simulink model "num2ASCIIsequenced_V2"  (Simulink 7.1)
settings: Solver=FixedStepDiscrete  StartTime=0.0  StopTime=.1  FixedStep=.0005  RelTol=1e-3
libraries: dsPICdrivers x6
settings Model: Creator=ij8977  LastModifiedBy=Lubin  ExtModeTrigDuration=10000
settings SolverCC: PositivePriorityOrder=on
settings OptimizationCC: InitFltsAndDblsToZero=off  OptimizeModelRefInitCode=on  LifeSpan=1
settings HardwareCC: ProdBitPerInt=16  ProdEndianess=LittleEndian  ProdWordSize=16  ProdHWDeviceType=16-bit Generic
settings RTWCC: SystemTargetFile=dspic.tlc  TemplateMakefile=dspic_pic30_gcc.tmf  PostCodeGenCommand=dsPIC_Compile()  Description=Embedded Target for Microchip dsPIC (real-time)  GenerateReport=on  ProcessScript=dspic_make_rtw_hook  IncludeHyperlinkInReport=on  LaunchReport=on  GenerateTraceInfo=on  GenerateTraceReport=on  GenerateTraceReportSl=on  GenerateTraceReportSf=on  GenerateTraceReportEml=on
settings CodeAppCC: IgnoreCustomStorageClasses=off
settings STFCustomTargetCC: ModelReferenceCompliant=off  IncludeMdlTerminateFcn=off  CombineOutputUpdateFcns=on  SuppressErrorStatus=on  ERTCustomFileBanners=on  SupportContinuousTime=off  SupportNonInlinedSFcns=off  SystemTargetFile=dspic.tlc
settings ERTTargetCC: ModelReferenceCompliant=off  ParMdlRefBuildCompliant=off  CompOptLevelCompliant=off  IncludeMdlTerminateFcn=off  SuppressErrorStatus=on  ERTFirstTimeCompliant=off  ModelStepFunctionPrototypeControlCompliant=off  CPPClassGenCompliant=off  ExtModeMexFile=noextcomm  InlinedParameterPlacement=NonHierarchical  ERTSrcFileBannerTemplate=dsPIC_code_template.cgt  ERTHdrFileBannerTemplate=dsPIC_code_template.cgt  ERTDataSrcFileTemplate=dsPIC_code_template.cgt  ERTDataHdrFileTemplate=dsPIC_code_template.cgt  ERTCustomFileTemplate=dsPIC_main.tlc
settings CustomProperty: DataType=string  Value=C:\PROGRA~1\MATLAB\R2010a\bin\win64\gmake

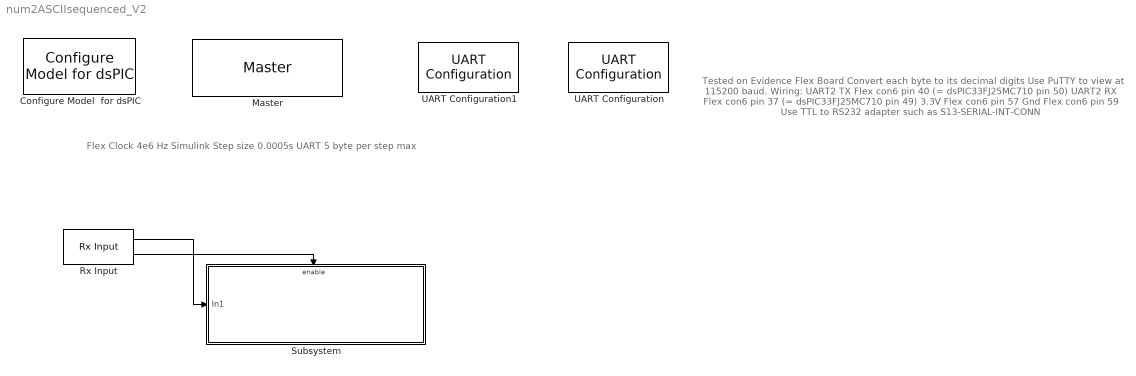
== system num2ASCIIsequenced_V2 ==
  note: Tested on Evidence Flex Board
      | Convert each byte to its decimal digits
      | Use PuTTY to view at 115200 baud.
      |
      | Wiring:
      | UART2 TX Flex con6 pin 40 (= dsPIC33FJ25MC710 pin 50)
      | UART2 RX Flex con6 pin 37 (= dsPIC33FJ25MC710 pin 49)
      | 3.3V Flex con6 pin 57
      | Gnd Flex con6 pin 59
      |
      | Use TTL to RS232 adapter such as S13-SERIAL-INT-CONN
  note: Flex Clock 4e6 Hz
      | Simulink Step size 0.0005s
      | UART 5 byte per step max
  Configure Model  for dsPIC : dsPICdrivers/Simulink Configuration/Configure Model  for dsPIC
  Master : dsPICdrivers/Master  Tag=dsPIC_MASTER  Priority=1  TimeStepType=Timer1  picType=33fJ256MC710  fcy=40000000  Quartz_33f=4e6  PLLActive_33f=on  fcyDesired_33f=40000000  tmr1="[1  19999  0]"  tmr1Info="Time Step : 0.0005  ;   Error : 0%  PR1=19999"  tmr2345="[0  0  0  0  0  0  0  0]"  tmr2345cfg=[-1 -1 -1 -1 -1 -1 -1 -1]  IOautoConf=on  typePort="[ 0  0  0  0  0  0  0  0  0  0  0  0  0  0  0  0  0  0  0  0  0  0  0  0  0  0  0  0  0  0  0  0  0  0  0  0  0  0  0  0  0  0  0  0  0  0  0  0  0  0  0  0  0  0  0  0  0  0  0  0  0  0  0  0  0  0  0  0  0  0  0  0  0  0  0  0  0  0  0  0  0  0  4  0  4  5  0  0  0  0  0  0  0  0  0  0  0  0  0  0  0  0  0  0  0  0  0  0  0  0  0  0 ]"  TRIS="[ 65535  65535  65535  65535  65535  65535  65535 ]"  ADPCFG=0  MasterBusyPort=None  MasterOverloadPort=None  FOSC=Quartz (XT - HS)  ClockSwitchMonitor=Both disabled  TempProtection_33f=TEMP_ON  FPBOR=<empty>  PWRT=disable  MCLR=<empty>  ICD=ICS_NONE  JTAGEN=JTAGEN_OFF  PowerSave=off  OverrideFcy=off  NewFcy=1e6  PR2345="[65535  65535  65535  65535  65535  65535  65535  65535]"
  Rx Input : dsPICdrivers/Serial PORT/Rx Input  Tag=dsPIC_RX  Priority=5  UART=1  SampleTime=-1  BlockingFctChk=off  OutputDefault=0  IsPresentFlagChk=on
  Subsystem : Subsystem
  UART Configuration : dsPICdrivers/Serial PORT/UART Configuration  Tag=dsPIC_config_UART  Priority=2  UART=2  proposed_BAUD=115200  ALT_TX_RX=on  InterruptTxWhen=When Transmit Buffer is empty  TXInterruptPri=1  TxBufferSize=32  TXEN=on  InterruptRxWhen=When a character is received  RXInterruptPri=2  RxBufferSize=32  BAUD=115200  UxBRG=21  Info="UxBRG = 21   ||  Real Baud : 113636   ||  % error : -1.3573  ||  max 5.6818 Bytes / Step"  RealBaud=0
  UART Configuration1 : dsPICdrivers/Serial PORT/UART Configuration  Tag=dsPIC_config_UART  Priority=2  UART=1  proposed_BAUD=115200  ALT_TX_RX=on  InterruptTxWhen=When Transmit Buffer is empty  TXInterruptPri=1  TxBufferSize=32  TXEN=off  InterruptRxWhen=When Receive Buffer is 3/4 full (contain 3 characters)  RXInterruptPri=2  RxBufferSize=32  BAUD=115200  UxBRG=21  Info="UxBRG = 21   ||  Real Baud : 113636   ||  % error : -1.3573  ||  max 5.6818 Bytes / Step"  RealBaud=0
  wires:
  Rx Input/1 -> Subsystem/1(In1)
  Rx Input/2 -> Subsystem/Enable

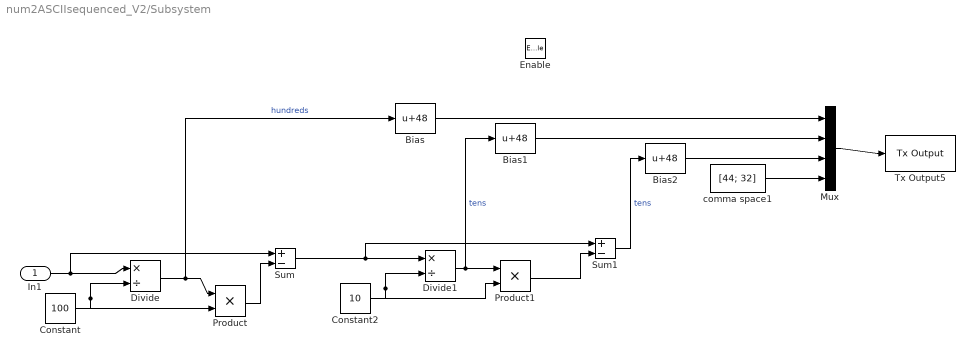
== system num2ASCIIsequenced_V2/Subsystem ==
  In1 : Inport
  Enable : EnablePort
  Bias : Bias  Bias=48
  Bias1 : Bias  Bias=48
  Bias2 : Bias  Bias=48
  Constant : Constant  Value=100  OutDataTypeMode=uint8  OutDataType=fixdt(1, 16)  OutScaling=2^0  OutDataTypeStr=uint8
  Constant2 : Constant  Value=10  OutDataTypeMode=uint8  OutDataType=fixdt(1, 16)  OutScaling=2^0  OutDataTypeStr=uint8
  Divide : Product  Inputs=*/  OutDataTypeMode=uint8  OutDataType=fixdt(1, 16)  OutScaling=2^-10  OutDataTypeStr=uint8
  Divide1 : Product  Inputs=*/  OutDataTypeMode=uint8  OutDataType=fixdt(1, 16)  OutScaling=2^-10  OutDataTypeStr=uint8
  Mux : Mux
  Product : Product  OutDataTypeMode=uint8  OutDataType=fixdt(1, 16)  OutScaling=2^0  OutDataTypeStr=uint8  RndMeth=Zero
  Product1 : Product  OutDataTypeMode=uint8  OutDataType=fixdt(1, 16)  OutScaling=2^0  OutDataTypeStr=uint8  RndMeth=Zero
  Sum : Sum  Inputs=+-  OutDataType=fixdt(1, 16)  OutScaling=2^0
  Sum1 : Sum  Inputs=+-  OutDataType=fixdt(1, 16)  OutScaling=2^0
  Tx Output5 : dsPICdrivers/Serial PORT/Tx Output  Tag=dsPIC_TX  Priority=5  UART=2  OrderingInOutPopup=None
  comma space1 : Constant  Value=[44; 32]  OutDataTypeMode=uint8  OutDataType=fixdt(1, 16)  OutScaling=2^0  OutDataTypeStr=uint8
  wires:
  In1/1 -> Sum/1, Divide/1
  Constant/1 -> Divide/2, Product/2
  Divide/1 -> Product/1, Bias/1  "hundreds"
  Product/1 -> Sum/2
  Sum/1 -> Sum1/1, Divide1/1
  Constant2/1 -> Product1/2, Divide1/2
  Divide1/1 -> Product1/1, Bias1/1  "tens"
  Product1/1 -> Sum1/2
  Sum1/1 -> Bias2/1  "tens"
  Bias/1 -> Mux/1
  Bias1/1 -> Mux/2
  Bias2/1 -> Mux/3
  comma space1/1 -> Mux/4
  Mux/1 -> Tx Output5/1
